simulink model "fw_io_in_hw"  (R2026b)
settings: Solver=VariableStepAuto
undefined symbols (not defined in the file or in its folder): CAN, diff, FD, P, Ts
libraries: simulink x40, stmutilitieslib x5, stm32blockslib x3, stm32h7xxblockslib x2, stm32f4xxblockslib x1, stm32IMUsensorslib x1
settings Model: Creator=aomar  LastModifiedBy=aomar

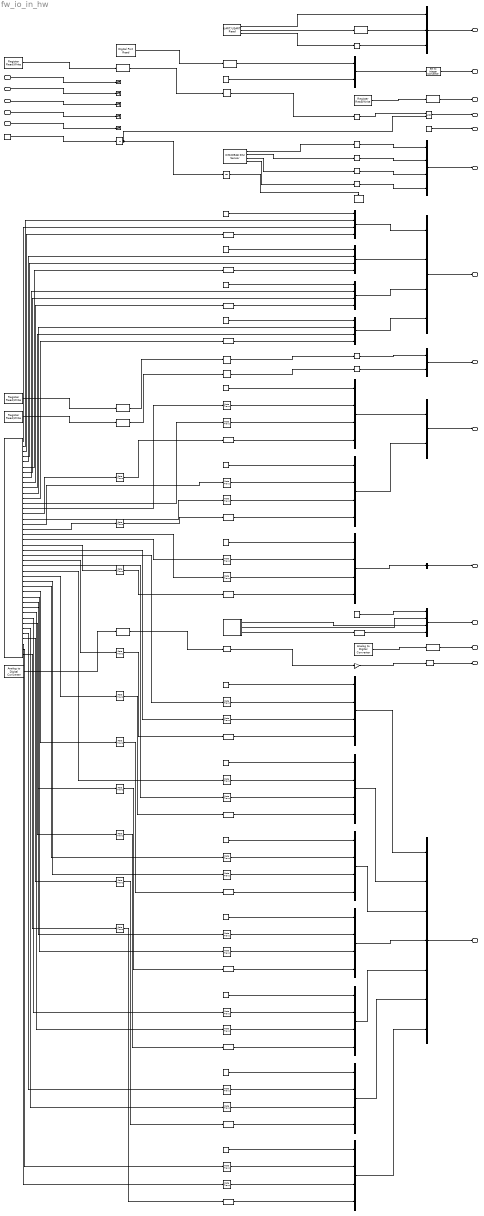
== system fw_io_in_hw ==
  in1k : Inport  OutDataTypeStr=Bus: Bus_McuIn1k  SampleTime=Ts.base
  in5 : Inport  Port=2  OutDataTypeStr=Bus: Bus_McuIn5  SampleTime=Ts.imu
  in10 : Inport  Port=3  OutDataTypeStr=Bus: Bus_McuIn10  SampleTime=Ts.ctrl
  in50 : Inport  Port=4  OutDataTypeStr=Bus: Bus_McuIn50  SampleTime=Ts.comm
  in100 : Inport  Port=5  OutDataTypeStr=Bus: Bus_McuIn100  SampleTime=Ts.hk
  ADC1_Conv : stm32h7xxblockslib/Analog to Digital Converter  ADCModule=ADC1  ConversionGroup=Regular  TriggerMode=Trigger and read  NumberOfConversions=8  EnableBufferConv=off  BufferLength=1  OutputStatus=off  SampleTime=Ts.comm  EnableSimPort=off  hoistedMaskSrc=ECSoC/ECSimCodegen/Analog to Digital Converter
  ADC1_u16 : DataTypeConversion  OutDataTypeStr=uint16  RndMeth=Round
  ADC3_TempSensor : stm32h7xxblockslib/Analog to Digital Converter  ADCModule=ADC3  ConversionGroup=Regular  TriggerMode=Trigger and read  NumberOfConversions=1  EnableBufferConv=off  BufferLength=1  OutputStatus=off  SampleTime=Ts.comm  EnableSimPort=off  hoistedMaskSrc=ECSoC/ECSimCodegen/Analog to Digital Converter
  ADC3_s : DataTypeConversion  OutDataTypeStr=single  RndMeth=Round
  BO1 : simulink/Logic and Bit Operations/Compare To Zero  relop=~=  OutDataTypeStr=boolean
  BO1_bit : simulink/Logic and Bit Operations/Bitwise Operator  logicop=AND  UseBitMask=on  BitMask=2^P.electronics.hw.fdcan_psr_bo_bit  BitMaskRealWorld=Stored Integer
  BO2 : simulink/Logic and Bit Operations/Compare To Zero  relop=~=  OutDataTypeStr=boolean
  BO2_bit : simulink/Logic and Bit Operations/Bitwise Operator  logicop=AND  UseBitMask=on  BitMask=2^P.electronics.hw.fdcan_psr_bo_bit  BitMaskRealWorld=Stored Integer
  BO_vec : Concatenate
  Bms_BC : BusCreator  Inputs=7  OutDataTypeStr=Bus: Bus_Can1_Bms  NonVirtualBus=on
      settings: InheritFromInputs=off
  Boot_false : Constant  Value=false  OutDataTypeStr=boolean  SampleTime=Ts.base
  CAN1_RX : Subsystem  TreatAsAtomicUnit=on  SystemSampleTime=Ts.ctrl
  CAN2_RX : Subsystem  TreatAsAtomicUnit=on  SystemSampleTime=Ts.comm
  DI_GPIOF : stm32f4xxblockslib/Digital Port Read  PortName=GPIOF  PinNumber=[0:13]  ReadOperation=on  IOAsArray=on  SampleTime=Ts.base  EnableSimPort=off  hoistedMaskSrc=ECSoC/ECSimCodegen/Digital Port Read
      settings: LibrarySourceBlock=stm32h7xxblockslib/Digital Port Read
  DI_bits : Concatenate
  DI_bool : DataTypeConversion  OutDataTypeStr=boolean  RndMeth=Round
  DI_pad : Constant  Value=false(1,16-P.electronics.hw.di_pins)  OutDataTypeStr=boolean  SampleTime=Ts.base
  DI_word : simulink/Logic and Bit Operations/Bit to Integer Converter  nbits=16  bitOrder=LSB first  signedOutputValues=Unsigned  outDtype=uint16  outDtypeSigned=Inherit via internal rule
      settings: LibrarySourceBlock=|
      | commutil2/Bit to Integer
      | Converter
  Esc_fast_BC : BusCreator  Inputs=4  OutDataTypeStr=Bus: Bus_Can1_EscFast  NonVirtualBus=on
      settings: InheritFromInputs=off
  Esc_slow_BC : BusCreator  Inputs=2  OutDataTypeStr=Bus: Bus_Can1_EscSlow  NonVirtualBus=on
      settings: InheritFromInputs=off
  FDCAN1_PSR : stmutilitieslib/Register Read//Write  Description=INTENDED (set in the T17 board setup): tgtHW 'STM32H7xx Based', devID 'STM32H743', regGrpName 'FDCAN1', regName 'PSR', opCode 'Read'.  tgtHW=STM32F4xx Based  devID=STM32F401  regGrpName=ADC_Common  regName=CSR  accessMode=Specified bits  opCode=Read  bitsToBeProcessed={ [ 15, 0 ] }  bitFields={'on','All';'off','OVR3';'off','STRT3';'off','JSTRT3';'off','JEOC3';'off','EOC3';'off','AWD3';'off','OVR2';'off','STRT2';'off','JSTRT2';'off','JEOC2';'off','EOC2';'off','AWD2';'off','OVR1';'off','STRT1';'off','JSTRT1';'off','JEOC1';'off','EOC1';'off','AWD1'}  SampleTime=1
  FDCAN2_PSR : stmutilitieslib/Register Read//Write  Description=INTENDED (set in the T17 board setup): tgtHW 'STM32H7xx Based', devID 'STM32H743', regGrpName 'FDCAN2', regName 'PSR', opCode 'Read'.  tgtHW=STM32F4xx Based  devID=STM32F401  regGrpName=ADC_Common  regName=CSR  accessMode=Specified bits  opCode=Read  bitsToBeProcessed={ [ 15, 0 ] }  bitFields={'on','All';'off','OVR3';'off','STRT3';'off','JSTRT3';'off','JEOC3';'off','EOC3';'off','AWD3';'off','OVR2';'off','STRT2';'off','JSTRT2';'off','JEOC2';'off','EOC2';'off','AWD2';'off','OVR1';'off','STRT1';'off','JSTRT1';'off','JEOC1';'off','EOC1';'off','AWD1'}  SampleTime=1
  First_tick : UnitDelay  InitialCondition=true  SampleTime=Ts.base
  Frame_alarm : BusCreator  Inputs=4  OutDataTypeStr=Bus: Bus_CanFrame8  NonVirtualBus=on
      settings: InheritFromInputs=off
  Frame_cells : BusCreator  Inputs=4  OutDataTypeStr=Bus: Bus_CanFrame8  NonVirtualBus=on
      settings: InheritFromInputs=off
  Frame_comp_cmd : BusCreator  Inputs=4  OutDataTypeStr=Bus: Bus_CanFrame64  NonVirtualBus=on
      settings: InheritFromInputs=off
  Frame_fb1_L : BusCreator  Inputs=4  OutDataTypeStr=Bus: Bus_CanFrame8  NonVirtualBus=on
      settings: InheritFromInputs=off
  Frame_fb1_R : BusCreator  Inputs=4  OutDataTypeStr=Bus: Bus_CanFrame8  NonVirtualBus=on
      settings: InheritFromInputs=off
  Frame_fb2_L : BusCreator  Inputs=4  OutDataTypeStr=Bus: Bus_CanFrame8  NonVirtualBus=on
      settings: InheritFromInputs=off
  Frame_fb2_R : BusCreator  Inputs=4  OutDataTypeStr=Bus: Bus_CanFrame8  NonVirtualBus=on
      settings: InheritFromInputs=off
  Frame_fb3_L : BusCreator  Inputs=4  OutDataTypeStr=Bus: Bus_CanFrame8  NonVirtualBus=on
      settings: InheritFromInputs=off
  Frame_fb3_R : BusCreator  Inputs=4  OutDataTypeStr=Bus: Bus_CanFrame8  NonVirtualBus=on
      settings: InheritFromInputs=off
  Frame_impl_fb : BusCreator  Inputs=4  OutDataTypeStr=Bus: Bus_CanFrame8  NonVirtualBus=on
      settings: InheritFromInputs=off
  Frame_limits : BusCreator  Inputs=4  OutDataTypeStr=Bus: Bus_CanFrame8  NonVirtualBus=on
      settings: InheritFromInputs=off
  Frame_power : BusCreator  Inputs=4  OutDataTypeStr=Bus: Bus_CanFrame8  NonVirtualBus=on
      settings: InheritFromInputs=off
  Frame_soc : BusCreator  Inputs=4  OutDataTypeStr=Bus: Bus_CanFrame8  NonVirtualBus=on
      settings: InheritFromInputs=off
  Frame_state : BusCreator  Inputs=4  OutDataTypeStr=Bus: Bus_CanFrame8  NonVirtualBus=on
      settings: InheritFromInputs=off
  Frame_vit : BusCreator  Inputs=4  OutDataTypeStr=Bus: Bus_CanFrame8  NonVirtualBus=on
      settings: InheritFromInputs=off
  ICM20948 : stm32IMUsensorslib/ICM20948 IMU Sensor  I2CModule=I2C1  I2CAddress=0x69  BitRate=400000  EnableDRDY=off  InterruptType=Active high  IsActiveAccel=on  IsActiveGyro=on  IsActiveMag=on  IsActiveTemp=on  IsActiveStatus=off  IsActiveTimeStamp=off  AccelerometerRange=+/-4g  AccelerometerODR=1125  AccelerometerBW=23.9 Hz  GyroscopeRange=+/-500 dps  GyroscopeODR=1125  GyroscopeBW=23.9 Hz  MagnetometerODR=100 Hz  TemperatureBW=34.1 Hz  DataType=single  SampleTime=Ts.imu  QueueSizeFactor=3
  IWDG1RSTF : simulink/Logic and Bit Operations/Bitwise Operator  logicop=AND  UseBitMask=on  BitMask=2^P.electronics.hw.rcc_rsr_iwdg1rstf_bit  BitMaskRealWorld=Stored Integer
  Id_alarm : Constant  Value=P.electronics.can.id.bms_alarm  OutDataTypeStr=uint32  SampleTime=Ts.hk
  Id_cells : Constant  Value=P.electronics.can.id.bms_cells  OutDataTypeStr=uint32  SampleTime=Ts.hk
  Id_comp_cmd : Constant  Value=P.electronics.can.id.comp_cmd  OutDataTypeStr=uint32  SampleTime=Ts.comm
  Id_fb1_L : Constant  Value=P.drive.can.id_fb1+1  OutDataTypeStr=uint32  SampleTime=Ts.ctrl
  Id_fb1_R : Constant  Value=P.drive.can.id_fb1+2  OutDataTypeStr=uint32  SampleTime=Ts.ctrl
  Id_fb2_L : Constant  Value=P.drive.can.id_fb2+1  OutDataTypeStr=uint32  SampleTime=Ts.comm
  Id_fb2_R : Constant  Value=P.drive.can.id_fb2+2  OutDataTypeStr=uint32  SampleTime=Ts.comm
  Id_fb3_L : Constant  Value=P.drive.can.id_fb3+1  OutDataTypeStr=uint32  SampleTime=Ts.ctrl
  Id_fb3_R : Constant  Value=P.drive.can.id_fb3+2  OutDataTypeStr=uint32  SampleTime=Ts.ctrl
  Id_impl_fb : Constant  Value=P.electronics.can.id.impl_fb  OutDataTypeStr=uint32  SampleTime=Ts.comm
  Id_limits : Constant  Value=P.electronics.can.id.bms_limits  OutDataTypeStr=uint32  SampleTime=Ts.hk
  Id_power : Constant  Value=P.electronics.can.id.bms_power  OutDataTypeStr=uint32  SampleTime=Ts.hk
  Id_soc : Constant  Value=P.electronics.can.id.bms_soc  OutDataTypeStr=uint32  SampleTime=Ts.hk
  Id_state : Constant  Value=P.electronics.can.id.bms_state  OutDataTypeStr=uint32  SampleTime=Ts.hk
  Id_vit : Constant  Value=P.electronics.can.id.bms_vit  OutDataTypeStr=uint32  SampleTime=Ts.hk
  Impl_BC : BusCreator  Inputs=1  OutDataTypeStr=Bus: Bus_Can1_Impl  NonVirtualBus=on
      settings: InheritFromInputs=off
  Imu_BC : BusCreator  Inputs=4  OutDataTypeStr=Bus: Bus_ImuRaw  NonVirtualBus=on
      settings: InheritFromInputs=off
  Imu_vec{1..4} (4 alike) : Reshape
  New_alarm : simulink/Logic and Bit Operations/Detect Change  vinit=0  OutDataTypeStr=boolean
  New_cells : simulink/Logic and Bit Operations/Detect Change  vinit=0  OutDataTypeStr=boolean
  New_comp_cmd : simulink/Logic and Bit Operations/Detect Change  vinit=0  OutDataTypeStr=boolean
  New_fb1_L : simulink/Logic and Bit Operations/Detect Change  vinit=0  OutDataTypeStr=boolean
  New_fb1_R : simulink/Logic and Bit Operations/Detect Change  vinit=0  OutDataTypeStr=boolean
  New_fb2_L : simulink/Logic and Bit Operations/Detect Change  vinit=0  OutDataTypeStr=boolean
  New_fb2_R : simulink/Logic and Bit Operations/Detect Change  vinit=0  OutDataTypeStr=boolean
  New_fb3_L : simulink/Logic and Bit Operations/Detect Change  vinit=0  OutDataTypeStr=boolean
  New_fb3_R : simulink/Logic and Bit Operations/Detect Change  vinit=0  OutDataTypeStr=boolean
  New_impl_fb : simulink/Logic and Bit Operations/Detect Change  vinit=0  OutDataTypeStr=boolean
  New_limits : simulink/Logic and Bit Operations/Detect Change  vinit=0  OutDataTypeStr=boolean
  New_power : simulink/Logic and Bit Operations/Detect Change  vinit=0  OutDataTypeStr=boolean
  New_soc : simulink/Logic and Bit Operations/Detect Change  vinit=0  OutDataTypeStr=boolean
  New_state : simulink/Logic and Bit Operations/Detect Change  vinit=0  OutDataTypeStr=boolean
  New_vit : simulink/Logic and Bit Operations/Detect Change  vinit=0  OutDataTypeStr=boolean
  No_inject : Constant  Value=0  OutDataTypeStr=uint32  SampleTime=Ts.base
  PSR1_u32 : DataTypeConversion  OutDataTypeStr=uint32  RndMeth=Round
  PSR2_u32 : DataTypeConversion  OutDataTypeStr=uint32  RndMeth=Round
  RCC_RSR : stmutilitieslib/Register Read//Write  Description=INTENDED (set in the T17 board setup): tgtHW 'STM32H7xx Based', devID 'STM32H743', regGrpName 'RCC', regName 'RSR', opCode 'Read'.  tgtHW=STM32F4xx Based  devID=STM32F401  regGrpName=ADC_Common  regName=CSR  accessMode=Specified bits  opCode=Read  bitsToBeProcessed={ [ 15, 0 ] }  bitFields={'on','All';'off','OVR3';'off','STRT3';'off','JSTRT3';'off','JEOC3';'off','EOC3';'off','AWD3';'off','OVR2';'off','STRT2';'off','JSTRT2';'off','JEOC2';'off','EOC2';'off','AWD2';'off','OVR1';'off','STRT1';'off','JSTRT1';'off','JEOC1';'off','EOC1';'off','AWD1'}  SampleTime=1
  RMVF_write : Subsystem
  RSR_u32 : DataTypeConversion  OutDataTypeStr=uint32  RndMeth=Round
  RT_alarm_1 : RateTransition  OutPortSampleTime=Ts.hk
  RT_alarm_2 : RateTransition  OutPortSampleTime=Ts.hk
  RT_alarm_3 : RateTransition  OutPortSampleTime=Ts.hk
  RT_cells_1 : RateTransition  OutPortSampleTime=Ts.hk
  RT_cells_2 : RateTransition  OutPortSampleTime=Ts.hk
  RT_cells_3 : RateTransition  OutPortSampleTime=Ts.hk
  RT_fb2_L_1 : RateTransition  OutPortSampleTime=Ts.comm
  RT_fb2_L_2 : RateTransition  OutPortSampleTime=Ts.comm
  RT_fb2_L_3 : RateTransition  OutPortSampleTime=Ts.comm
  RT_fb2_R_1 : RateTransition  OutPortSampleTime=Ts.comm
  RT_fb2_R_2 : RateTransition  OutPortSampleTime=Ts.comm
  RT_fb2_R_3 : RateTransition  OutPortSampleTime=Ts.comm
  RT_impl_fb_1 : RateTransition  OutPortSampleTime=Ts.comm
  RT_impl_fb_2 : RateTransition  OutPortSampleTime=Ts.comm
  RT_impl_fb_3 : RateTransition  OutPortSampleTime=Ts.comm
  RT_limits_1 : RateTransition  OutPortSampleTime=Ts.hk
  RT_limits_2 : RateTransition  OutPortSampleTime=Ts.hk
  RT_limits_3 : RateTransition  OutPortSampleTime=Ts.hk
  RT_power_1 : RateTransition  OutPortSampleTime=Ts.hk
  RT_power_2 : RateTransition  OutPortSampleTime=Ts.hk
  RT_power_3 : RateTransition  OutPortSampleTime=Ts.hk
  RT_soc_1 : RateTransition  OutPortSampleTime=Ts.hk
  RT_soc_2 : RateTransition  OutPortSampleTime=Ts.hk
  RT_soc_3 : RateTransition  OutPortSampleTime=Ts.hk
  RT_state_1 : RateTransition  OutPortSampleTime=Ts.hk
  RT_state_2 : RateTransition  OutPortSampleTime=Ts.hk
  RT_state_3 : RateTransition  OutPortSampleTime=Ts.hk
  RT_vit_1 : RateTransition  OutPortSampleTime=Ts.hk
  RT_vit_2 : RateTransition  OutPortSampleTime=Ts.hk
  RT_vit_3 : RateTransition  OutPortSampleTime=Ts.hk
  Reset_at_boot : Logic  AllPortsSameDT=off  OutDataTypeStr=boolean
  Rst_seen : simulink/Logic and Bit Operations/Compare To Zero  relop=~=  OutDataTypeStr=boolean
  SBUS_UART : stm32blockslib/UART//USART Read  UARTModule=USART2  DataType=uint8  DataLength=32  BlockingMode=off  BlockingTimeout=0.1  OutputLength=on  OutputStatus=on  SampleTime=Ts.base
      settings: LibrarySourceBlock=stm32h7xxblockslib/UART//USART Read
  Sbus_BC : BusCreator  Inputs=3  OutDataTypeStr=Bus: Bus_SbusStream  NonVirtualBus=on
      settings: InheritFromInputs=off
  Second_tick : UnitDelay  InitialCondition=false  SampleTime=Ts.base
  TIM2_CNT : stmutilitieslib/Register Read//Write  Description=INTENDED (set in the T17 board setup): tgtHW 'STM32H7xx Based', devID 'STM32H743', regGrpName 'TIM2', regName 'CNT', opCode 'Read'.  tgtHW=STM32F4xx Based  devID=STM32F401  regGrpName=ADC_Common  regName=CSR  accessMode=Specified bits  opCode=Read  bitsToBeProcessed={ [ 15, 0 ] }  bitFields={'on','All';'off','OVR3';'off','STRT3';'off','JSTRT3';'off','JEOC3';'off','EOC3';'off','AWD3';'off','OVR2';'off','STRT2';'off','JSTRT2';'off','JEOC2';'off','EOC2';'off','AWD2';'off','OVR1';'off','STRT1';'off','JSTRT1';'off','JEOC1';'off','EOC1';'off','AWD1'}  SampleTime=1
  TS_T1 : Bias  Bias=P.electronics.adc.ts_cal_T(1)  SaturateOnIntegerOverflow=off
  TS_c1 : Bias  Bias=-P.electronics.adc.ts_cal_cnt(1)  SaturateOnIntegerOverflow=off
  TS_slope : Gain  Gain=diff(P.electronics.adc.ts_cal_T)/diff(P.electronics.adc.ts_cal_cnt)
  T_in{5,10,50,100} (4 alike) : Terminator
  T_in1k : Terminator
  T_us_u32 : DataTypeConversion  OutDataTypeStr=uint32  RndMeth=Round
  Uart_err : simulink/Logic and Bit Operations/Compare To Zero  relop=~=  OutDataTypeStr=boolean
  Uart_len : DataTypeConversion  OutDataTypeStr=uint8  RndMeth=Round
  sbus : Outport  OutDataTypeStr=Bus: Bus_SbusStream
  di_word : Outport  Port=2  OutDataTypeStr=uint16
  t_us : Outport  Port=3  OutDataTypeStr=uint32
  reset_flag : Outport  Port=4  OutDataTypeStr=boolean
  fault_inject : Outport  Port=5  OutDataTypeStr=uint32
  imu : Outport  Port=6  OutDataTypeStr=Bus: Bus_ImuRaw
  can1_esc : Outport  Port=7  OutDataTypeStr=Bus: Bus_Can1_EscFast
  busoff : Outport  Port=8  OutDataTypeStr=boolean
  can1_escslow : Outport  Port=9  OutDataTypeStr=Bus: Bus_Can1_EscSlow
  can1_impl : Outport  Port=10  OutDataTypeStr=Bus: Bus_Can1_Impl
  can2_comp : Outport  Port=11  OutDataTypeStr=Bus: Bus_CanFrame64
  adc_raw : Outport  Port=12  OutDataTypeStr=uint16
  mcu_temp_degC : Outport  Port=13  OutDataTypeStr=single
  can1_bms : Outport  Port=14  OutDataTypeStr=Bus: Bus_Can1_Bms
  wires:
  in1k/1 -> T_in1k/1  "in1k"
  in5/1 -> T_in5/1  "in5"
  in10/1 -> T_in10/1  "in10"
  in50/1 -> T_in50/1  "in50"
  in100/1 -> T_in100/1  "in100"
  Boot_false/1 -> First_tick/1  "Boot_false"
  RCC_RSR/1 -> RSR_u32/1  "RCC_RSR"
  FDCAN1_PSR/1 -> PSR1_u32/1  "FDCAN1_PSR"
  FDCAN2_PSR/1 -> PSR2_u32/1  "FDCAN2_PSR"
  CAN1_RX/1(data_fb1_L) -> Frame_fb1_L/3  "data"
  CAN1_RX/2(len_fb1_L) -> Frame_fb1_L/2  "len"
  CAN1_RX/3(cnt_fb1_L) -> New_fb1_L/1  "cnt_fb1_L"
  CAN1_RX/4(data_fb1_R) -> Frame_fb1_R/3  "data"
  CAN1_RX/5(len_fb1_R) -> Frame_fb1_R/2  "len"
  CAN1_RX/6(cnt_fb1_R) -> New_fb1_R/1  "cnt_fb1_R"
  CAN1_RX/7(data_fb3_L) -> Frame_fb3_L/3  "data"
  CAN1_RX/8(len_fb3_L) -> Frame_fb3_L/2  "len"
  CAN1_RX/9(cnt_fb3_L) -> New_fb3_L/1  "cnt_fb3_L"
  CAN1_RX/10(data_fb3_R) -> Frame_fb3_R/3  "data"
  CAN1_RX/11(len_fb3_R) -> Frame_fb3_R/2  "len"
  CAN1_RX/12(cnt_fb3_R) -> New_fb3_R/1  "cnt_fb3_R"
  CAN1_RX/13(data_fb2_L) -> RT_fb2_L_1/1  "CAN1_RX_13"
  CAN1_RX/14(len_fb2_L) -> RT_fb2_L_2/1  "CAN1_RX_14"
  CAN1_RX/15(cnt_fb2_L) -> RT_fb2_L_3/1  "CAN1_RX_15"
  CAN1_RX/16(data_fb2_R) -> RT_fb2_R_1/1  "CAN1_RX_16"
  CAN1_RX/17(len_fb2_R) -> RT_fb2_R_2/1  "CAN1_RX_17"
  CAN1_RX/18(cnt_fb2_R) -> RT_fb2_R_3/1  "CAN1_RX_18"
  CAN1_RX/19(data_impl_fb) -> RT_impl_fb_1/1  "CAN1_RX_19"
  CAN1_RX/20(len_impl_fb) -> RT_impl_fb_2/1  "CAN1_RX_20"
  CAN1_RX/21(cnt_impl_fb) -> RT_impl_fb_3/1  "CAN1_RX_21"
  CAN1_RX/22(data_limits) -> RT_limits_1/1  "CAN1_RX_22"
  CAN1_RX/23(len_limits) -> RT_limits_2/1  "CAN1_RX_23"
  CAN1_RX/24(cnt_limits) -> RT_limits_3/1  "CAN1_RX_24"
  CAN1_RX/25(data_soc) -> RT_soc_1/1  "CAN1_RX_25"
  CAN1_RX/26(len_soc) -> RT_soc_2/1  "CAN1_RX_26"
  CAN1_RX/27(cnt_soc) -> RT_soc_3/1  "CAN1_RX_27"
  CAN1_RX/28(data_vit) -> RT_vit_1/1  "CAN1_RX_28"
  CAN1_RX/29(len_vit) -> RT_vit_2/1  "CAN1_RX_29"
  CAN1_RX/30(cnt_vit) -> RT_vit_3/1  "CAN1_RX_30"
  CAN1_RX/31(data_alarm) -> RT_alarm_1/1  "CAN1_RX_31"
  CAN1_RX/32(len_alarm) -> RT_alarm_2/1  "CAN1_RX_32"
  CAN1_RX/33(cnt_alarm) -> RT_alarm_3/1  "CAN1_RX_33"
  CAN1_RX/34(data_cells) -> RT_cells_1/1  "CAN1_RX_34"
  CAN1_RX/35(len_cells) -> RT_cells_2/1  "CAN1_RX_35"
  CAN1_RX/36(cnt_cells) -> RT_cells_3/1  "CAN1_RX_36"
  CAN1_RX/37(data_state) -> RT_state_1/1  "CAN1_RX_37"
  CAN1_RX/38(len_state) -> RT_state_2/1  "CAN1_RX_38"
  CAN1_RX/39(cnt_state) -> RT_state_3/1  "CAN1_RX_39"
  CAN1_RX/40(data_power) -> RT_power_1/1  "CAN1_RX_40"
  CAN1_RX/41(len_power) -> RT_power_2/1  "CAN1_RX_41"
  CAN1_RX/42(cnt_power) -> RT_power_3/1  "CAN1_RX_42"
  ADC3_TempSensor/1 -> ADC3_s/1  "ADC3_TempSensor"
  First_tick/1 -> Second_tick/1, Reset_at_boot/2  "first_tick"
  RT_fb2_L_3/1 -> New_fb2_L/1  "cnt_fb2_L"
  RT_fb2_R_3/1 -> New_fb2_R/1  "cnt_fb2_R"
  RT_impl_fb_3/1 -> New_impl_fb/1  "cnt_impl_fb"
  RT_limits_3/1 -> New_limits/1  "cnt_limits"
  RT_soc_3/1 -> New_soc/1  "cnt_soc"
  RT_vit_3/1 -> New_vit/1  "cnt_vit"
  RT_alarm_3/1 -> New_alarm/1  "cnt_alarm"
  RT_cells_3/1 -> New_cells/1  "cnt_cells"
  RT_state_3/1 -> New_state/1  "cnt_state"
  RT_power_3/1 -> New_power/1  "cnt_power"
  RSR_u32/1 -> IWDG1RSTF/1  "RSR_u32"
  PSR1_u32/1 -> BO1_bit/1  "PSR1_u32"
  PSR2_u32/1 -> BO2_bit/1  "PSR2_u32"
  ADC3_s/1 -> TS_c1/1  "ADC3_s"
  DI_GPIOF/1 -> DI_bool/1  "DI_GPIOF"
  DI_pad/1 -> DI_bits/2  "DI_pad"
  Id_fb1_L/1 -> Frame_fb1_L/1  "id"
  Id_fb1_R/1 -> Frame_fb1_R/1  "id"
  Id_fb3_L/1 -> Frame_fb3_L/1  "id"
  Id_fb3_R/1 -> Frame_fb3_R/1  "id"
  Id_fb2_L/1 -> Frame_fb2_L/1  "id"
  Id_fb2_R/1 -> Frame_fb2_R/1  "id"
  Id_impl_fb/1 -> Frame_impl_fb/1  "id"
  Id_limits/1 -> Frame_limits/1  "id"
  Id_soc/1 -> Frame_soc/1  "id"
  Id_vit/1 -> Frame_vit/1  "id"
  Id_alarm/1 -> Frame_alarm/1  "id"
  Id_cells/1 -> Frame_cells/1  "id"
  Id_state/1 -> Frame_state/1  "id"
  Id_power/1 -> Frame_power/1  "id"
  Second_tick/1 -> RMVF_write/Enable  "second_tick"
  IWDG1RSTF/1 -> Rst_seen/1  "IWDG1RSTF"
  BO1_bit/1 -> BO1/1  "BO1_bit"
  BO2_bit/1 -> BO2/1  "BO2_bit"
  RT_fb2_L_2/1 -> Frame_fb2_L/2  "len"
  RT_fb2_L_1/1 -> Frame_fb2_L/3  "data"
  RT_fb2_R_2/1 -> Frame_fb2_R/2  "len"
  RT_fb2_R_1/1 -> Frame_fb2_R/3  "data"
  RT_impl_fb_2/1 -> Frame_impl_fb/2  "len"
  RT_impl_fb_1/1 -> Frame_impl_fb/3  "data"
  TS_c1/1 -> TS_slope/1  "TS_c1"
  RT_limits_2/1 -> Frame_limits/2  "len"
  RT_limits_1/1 -> Frame_limits/3  "data"
  RT_soc_2/1 -> Frame_soc/2  "len"
  RT_soc_1/1 -> Frame_soc/3  "data"
  RT_vit_2/1 -> Frame_vit/2  "len"
  RT_vit_1/1 -> Frame_vit/3  "data"
  RT_alarm_2/1 -> Frame_alarm/2  "len"
  RT_alarm_1/1 -> Frame_alarm/3  "data"
  RT_cells_2/1 -> Frame_cells/2  "len"
  RT_cells_1/1 -> Frame_cells/3  "data"
  RT_state_2/1 -> Frame_state/2  "len"
  RT_state_1/1 -> Frame_state/3  "data"
  RT_power_2/1 -> Frame_power/2  "len"
  RT_power_1/1 -> Frame_power/3  "data"
  New_fb1_L/1 -> Frame_fb1_L/4  "valid"
  New_fb1_R/1 -> Frame_fb1_R/4  "valid"
  New_fb3_L/1 -> Frame_fb3_L/4  "valid"
  New_fb3_R/1 -> Frame_fb3_R/4  "valid"
  New_fb2_L/1 -> Frame_fb2_L/4  "valid"
  New_fb2_R/1 -> Frame_fb2_R/4  "valid"
  New_impl_fb/1 -> Frame_impl_fb/4  "valid"
  New_limits/1 -> Frame_limits/4  "valid"
  New_soc/1 -> Frame_soc/4  "valid"
  New_vit/1 -> Frame_vit/4  "valid"
  New_alarm/1 -> Frame_alarm/4  "valid"
  New_cells/1 -> Frame_cells/4  "valid"
  New_state/1 -> Frame_state/4  "valid"
  New_power/1 -> Frame_power/4  "valid"
  DI_bool/1 -> DI_bits/1  "DI_bool"
  SBUS_UART/1 -> Sbus_BC/1  "bytes"
  SBUS_UART/2 -> Uart_len/1  "SBUS_UART_2"
  SBUS_UART/3 -> Uart_err/1  "SBUS_UART_3"
  CAN2_RX/1(data_comp_cmd) -> Frame_comp_cmd/3  "data"
  CAN2_RX/2(len_comp_cmd) -> Frame_comp_cmd/2  "len"
  CAN2_RX/3(cnt_comp_cmd) -> New_comp_cmd/1  "cnt_comp_cmd"
  ICM20948/1 -> Imu_vec1/1  "ICM20948_1"
  ICM20948/2 -> Imu_vec2/1  "ICM20948_2"
  ICM20948/3 -> Imu_vec3/1  "ICM20948_3"
  ICM20948/4 -> Imu_vec4/1  "ICM20948_4"
  DI_bits/1 -> DI_word/1  "DI_bits"
  Frame_fb1_L/1 -> Esc_fast_BC/1  "fb1_L"
  Frame_fb1_R/1 -> Esc_fast_BC/2  "fb1_R"
  Frame_fb3_L/1 -> Esc_fast_BC/3  "fb3_L"
  Frame_fb3_R/1 -> Esc_fast_BC/4  "fb3_R"
  Frame_fb2_L/1 -> Esc_slow_BC/1  "fb2_L"
  Frame_fb2_R/1 -> Esc_slow_BC/2  "fb2_R"
  Frame_impl_fb/1 -> Impl_BC/1  "impl_fb"
  Frame_limits/1 -> Bms_BC/1  "limits"
  Frame_soc/1 -> Bms_BC/2  "soc"
  Frame_vit/1 -> Bms_BC/3  "vit"
  Frame_alarm/1 -> Bms_BC/4  "alarm"
  Frame_cells/1 -> Bms_BC/5  "cells"
  Frame_state/1 -> Bms_BC/6  "state"
  Frame_power/1 -> Bms_BC/7  "power"
  Uart_err/1 -> Sbus_BC/3  "uart_err"
  Rst_seen/1 -> Reset_at_boot/1  "Rst_seen"
  Imu_vec1/1 -> Imu_BC/1  "Acceleration"
  Imu_vec2/1 -> Imu_BC/2  "AngularRate"
  Imu_vec3/1 -> Imu_BC/3  "MagneticField"
  Imu_vec4/1 -> Imu_BC/4  "Temperature"
  BO1/1 -> BO_vec/1  "can1_busoff"
  BO2/1 -> BO_vec/2  "can2_busoff"
  Id_comp_cmd/1 -> Frame_comp_cmd/1  "id"
  TS_slope/1 -> TS_T1/1  "TS_slope"
  New_comp_cmd/1 -> Frame_comp_cmd/4  "valid"
  Uart_len/1 -> Sbus_BC/2  "len"
  TIM2_CNT/1 -> T_us_u32/1  "TIM2_CNT"
  ADC1_Conv/1 -> ADC1_u16/1  "ADC1_Conv"
  Sbus_BC/1 -> sbus/1  "sbus"
  Imu_BC/1 -> imu/1  "imu"
  Esc_fast_BC/1 -> can1_esc/1  "can1_esc"
  BO_vec/1 -> busoff/1  "busoff"
  Esc_slow_BC/1 -> can1_escslow/1  "can1_escslow"
  Impl_BC/1 -> can1_impl/1  "can1_impl"
  Frame_comp_cmd/1 -> can2_comp/1  "can2_comp"
  Bms_BC/1 -> can1_bms/1  "can1_bms"
  Reset_at_boot/1 -> reset_flag/1  "reset_flag"
  No_inject/1 -> fault_inject/1  "fault_inject"
  TS_T1/1 -> mcu_temp_degC/1  "mcu_temp_degC"
  T_us_u32/1 -> t_us/1  "t_us"
  ADC1_u16/1 -> adc_raw/1  "adc_raw"
  DI_word/1 -> di_word/1  "di_word"

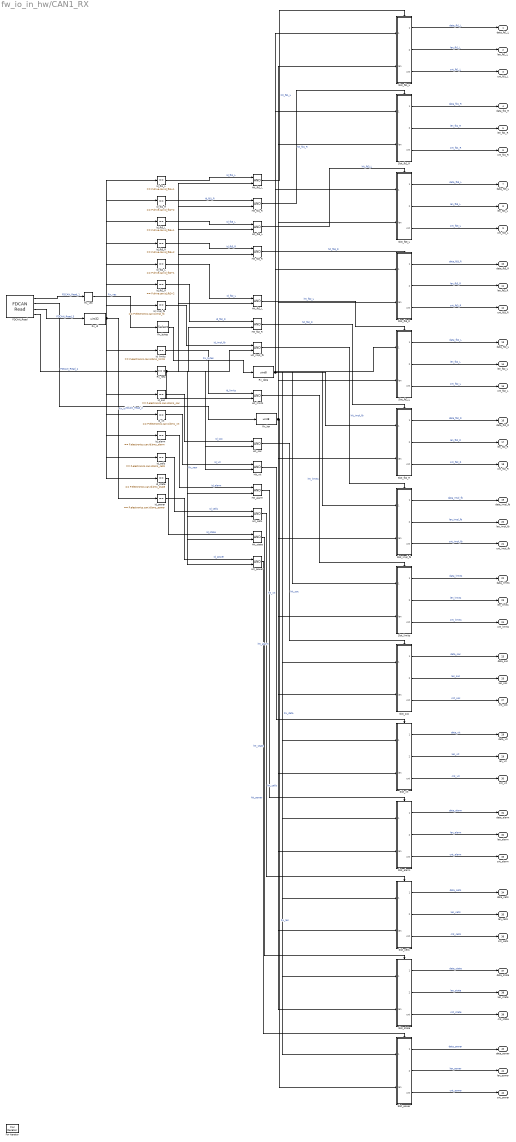
== system fw_io_in_hw/CAN1_RX ==
  FDCAN_Read : stm32blockslib/FDCAN Read  FDCANModule=FDCAN1  BlockMode=Receive  OperationReadMode=Data  OperationWriteMode=Data  ReadSource=FIFO 0  BufferNumber=0  OutputTypeReadMode=Unpacked  DataFormatWriteMode=Raw data  CANFrameType=CAN  IdentifierTypeVia=Dialog  IdentifierType=Standard (11-bit identifier)  IdentifierVia=Inport  Identifier=100  DataLengthVia=Inport  DataLength=64  OutputIdType=off  IsBitRateSwitchingEnabled=off  TransmitRemoteFrame=off  OutputFrameType=off  OutputBRS=off  OutputRemoteFrame=off  OutputTxFifoLevel=off  OutputRxFifoLevel=off  OutputStatus=on  Timeout=0.001  SampleTime=-1
      settings: LibrarySourceBlock=stm32h7xxblockslib/FDCAN Read
  For Iterator : ForIterator  IterationLimit=P.electronics.hw.can1_rx_iter  ShowIterationPort=off
  Hit_alarm : Logic  AllPortsSameDT=off  OutDataTypeStr=boolean
  Hit_cells : Logic  AllPortsSameDT=off  OutDataTypeStr=boolean
  Hit_fb1_L : Logic  AllPortsSameDT=off  OutDataTypeStr=boolean
  Hit_fb1_R : Logic  AllPortsSameDT=off  OutDataTypeStr=boolean
  Hit_fb2_L : Logic  AllPortsSameDT=off  OutDataTypeStr=boolean
  Hit_fb2_R : Logic  AllPortsSameDT=off  OutDataTypeStr=boolean
  Hit_fb3_L : Logic  AllPortsSameDT=off  OutDataTypeStr=boolean
  Hit_fb3_R : Logic  AllPortsSameDT=off  OutDataTypeStr=boolean
  Hit_impl_fb : Logic  AllPortsSameDT=off  OutDataTypeStr=boolean
  Hit_limits : Logic  AllPortsSameDT=off  OutDataTypeStr=boolean
  Hit_power : Logic  AllPortsSameDT=off  OutDataTypeStr=boolean
  Hit_soc : Logic  AllPortsSameDT=off  OutDataTypeStr=boolean
  Hit_state : Logic  AllPortsSameDT=off  OutDataTypeStr=boolean
  Hit_vit : Logic  AllPortsSameDT=off  OutDataTypeStr=boolean
  Id_alarm : simulink/Logic and Bit Operations/Compare To Constant  relop===  const=P.electronics.can.id.bms_alarm  OutDataTypeStr=boolean
  Id_cells : simulink/Logic and Bit Operations/Compare To Constant  relop===  const=P.electronics.can.id.bms_cells  OutDataTypeStr=boolean
  Id_fb1_L : simulink/Logic and Bit Operations/Compare To Constant  relop===  const=P.drive.can.id_fb1+1  OutDataTypeStr=boolean
  Id_fb1_R : simulink/Logic and Bit Operations/Compare To Constant  relop===  const=P.drive.can.id_fb1+2  OutDataTypeStr=boolean
  Id_fb2_L : simulink/Logic and Bit Operations/Compare To Constant  relop===  const=P.drive.can.id_fb2+1  OutDataTypeStr=boolean
  Id_fb2_R : simulink/Logic and Bit Operations/Compare To Constant  relop===  const=P.drive.can.id_fb2+2  OutDataTypeStr=boolean
  Id_fb3_L : simulink/Logic and Bit Operations/Compare To Constant  relop===  const=P.drive.can.id_fb3+1  OutDataTypeStr=boolean
  Id_fb3_R : simulink/Logic and Bit Operations/Compare To Constant  relop===  const=P.drive.can.id_fb3+2  OutDataTypeStr=boolean
  Id_impl_fb : simulink/Logic and Bit Operations/Compare To Constant  relop===  const=P.electronics.can.id.impl_fb  OutDataTypeStr=boolean
  Id_limits : simulink/Logic and Bit Operations/Compare To Constant  relop===  const=P.electronics.can.id.bms_limits  OutDataTypeStr=boolean
  Id_power : simulink/Logic and Bit Operations/Compare To Constant  relop===  const=P.electronics.can.id.bms_power  OutDataTypeStr=boolean
  Id_soc : simulink/Logic and Bit Operations/Compare To Constant  relop===  const=P.electronics.can.id.bms_soc  OutDataTypeStr=boolean
  Id_state : simulink/Logic and Bit Operations/Compare To Constant  relop===  const=P.electronics.can.id.bms_state  OutDataTypeStr=boolean
  Id_vit : simulink/Logic and Bit Operations/Compare To Constant  relop===  const=P.electronics.can.id.bms_vit  OutDataTypeStr=boolean
  Rx_bytes : Selector  IndexOptions=Index vector (dialog)  Indices=1:8  OutputSizes=1
  Rx_data : DataTypeConversion  OutDataTypeStr=uint8  RndMeth=Round
  Rx_id : DataTypeConversion  OutDataTypeStr=uint32  RndMeth=Round
  Rx_len : DataTypeConversion  OutDataTypeStr=uint8  RndMeth=Round
  Rx_new : simulink/Logic and Bit Operations/Compare To Zero  relop===  OutDataTypeStr=boolean
  Rx_vec : Reshape
  Slot_alarm : Subsystem
  Slot_cells : Subsystem
  Slot_fb1_L : Subsystem
  Slot_fb1_R : Subsystem
  Slot_fb2_L : Subsystem
  Slot_fb2_R : Subsystem
  Slot_fb3_L : Subsystem
  Slot_fb3_R : Subsystem
  Slot_impl_fb : Subsystem
  Slot_limits : Subsystem
  Slot_power : Subsystem
  Slot_soc : Subsystem
  Slot_state : Subsystem
  Slot_vit : Subsystem
  data_fb1_L : Outport
  len_fb1_L : Outport  Port=2
  cnt_fb1_L : Outport  Port=3
  data_fb1_R : Outport  Port=4
  len_fb1_R : Outport  Port=5
  cnt_fb1_R : Outport  Port=6
  data_fb3_L : Outport  Port=7
  len_fb3_L : Outport  Port=8
  cnt_fb3_L : Outport  Port=9
  data_fb3_R : Outport  Port=10
  len_fb3_R : Outport  Port=11
  cnt_fb3_R : Outport  Port=12
  data_fb2_L : Outport  Port=13
  len_fb2_L : Outport  Port=14
  cnt_fb2_L : Outport  Port=15
  data_fb2_R : Outport  Port=16
  len_fb2_R : Outport  Port=17
  cnt_fb2_R : Outport  Port=18
  data_impl_fb : Outport  Port=19
  len_impl_fb : Outport  Port=20
  cnt_impl_fb : Outport  Port=21
  data_limits : Outport  Port=22
  len_limits : Outport  Port=23
  cnt_limits : Outport  Port=24
  data_soc : Outport  Port=25
  len_soc : Outport  Port=26
  cnt_soc : Outport  Port=27
  data_vit : Outport  Port=28
  len_vit : Outport  Port=29
  cnt_vit : Outport  Port=30
  data_alarm : Outport  Port=31
  len_alarm : Outport  Port=32
  cnt_alarm : Outport  Port=33
  data_cells : Outport  Port=34
  len_cells : Outport  Port=35
  cnt_cells : Outport  Port=36
  data_state : Outport  Port=37
  len_state : Outport  Port=38
  cnt_state : Outport  Port=39
  data_power : Outport  Port=40
  len_power : Outport  Port=41
  cnt_power : Outport  Port=42
  wires:
  FDCAN_Read/1 -> Rx_vec/1  "FDCAN_Read_1"
  FDCAN_Read/2 -> Rx_len/1  "FDCAN_Read_2"
  FDCAN_Read/3 -> Rx_id/1  "FDCAN_Read_3"
  FDCAN_Read/4 -> Rx_new/1  "FDCAN_Read_4"
  Rx_vec/1 -> Rx_bytes/1  "Rx_vec"
  Rx_id/1 -> Id_power/1, Id_state/1, Id_fb1_L/1, Id_cells/1, Id_fb1_R/1, Id_alarm/1, Id_fb3_L/1, Id_vit/1, Id_fb3_R/1, Id_soc/1, Id_fb2_L/1, Id_fb2_R/1, Id_limits/1, Id_impl_fb/1  "Rx_id"
  Id_fb1_L/1 -> Hit_fb1_L/1  "Id_fb1_L"
  Id_fb1_R/1 -> Hit_fb1_R/1  "Id_fb1_R"
  Id_fb3_L/1 -> Hit_fb3_L/1  "Id_fb3_L"
  Id_fb3_R/1 -> Hit_fb3_R/1  "Id_fb3_R"
  Id_fb2_L/1 -> Hit_fb2_L/1  "Id_fb2_L"
  Id_fb2_R/1 -> Hit_fb2_R/1  "Id_fb2_R"
  Id_impl_fb/1 -> Hit_impl_fb/1  "Id_impl_fb"
  Id_limits/1 -> Hit_limits/1  "Id_limits"
  Rx_new/1 -> Hit_power/2, Hit_fb1_L/2, Hit_state/2, Hit_fb1_R/2, Hit_cells/2, Hit_fb3_L/2, Hit_alarm/2, Hit_fb3_R/2, Hit_vit/2, Hit_soc/2, Hit_fb2_L/2, Hit_fb2_R/2, Hit_limits/2, Hit_impl_fb/2  "Rx_new"
  Id_soc/1 -> Hit_soc/1  "Id_soc"
  Id_vit/1 -> Hit_vit/1  "Id_vit"
  Id_alarm/1 -> Hit_alarm/1  "Id_alarm"
  Id_cells/1 -> Hit_cells/1  "Id_cells"
  Id_state/1 -> Hit_state/1  "Id_state"
  Id_power/1 -> Hit_power/1  "Id_power"
  Rx_bytes/1 -> Rx_data/1  "Rx_bytes"
  Hit_fb1_L/1 -> Slot_fb1_L/Enable  "hit_fb1_L"
  Hit_fb1_R/1 -> Slot_fb1_R/Enable  "hit_fb1_R"
  Hit_fb3_L/1 -> Slot_fb3_L/Enable  "hit_fb3_L"
  Hit_fb3_R/1 -> Slot_fb3_R/Enable  "hit_fb3_R"
  Hit_fb2_L/1 -> Slot_fb2_L/Enable  "hit_fb2_L"
  Hit_fb2_R/1 -> Slot_fb2_R/Enable  "hit_fb2_R"
  Hit_impl_fb/1 -> Slot_impl_fb/Enable  "hit_impl_fb"
  Hit_limits/1 -> Slot_limits/Enable  "hit_limits"
  Hit_soc/1 -> Slot_soc/Enable  "hit_soc"
  Hit_vit/1 -> Slot_vit/Enable  "hit_vit"
  Hit_alarm/1 -> Slot_alarm/Enable  "hit_alarm"
  Hit_cells/1 -> Slot_cells/Enable  "hit_cells"
  Hit_state/1 -> Slot_state/Enable  "hit_state"
  Hit_power/1 -> Slot_power/Enable  "hit_power"
  Rx_data/1 -> Slot_power/1(data), Slot_state/1(data), Slot_cells/1(data), Slot_alarm/1(data), Slot_vit/1(data), Slot_fb1_L/1(data), Slot_soc/1(data), Slot_fb1_R/1(data), Slot_limits/1(data), Slot_fb3_L/1(data), Slot_impl_fb/1(data), Slot_fb3_R/1(data), Slot_fb2_R/1(data), Slot_fb2_L/1(data)  "Rx_data"
  Rx_len/1 -> Slot_power/2(len), Slot_state/2(len), Slot_cells/2(len), Slot_alarm/2(len), Slot_vit/2(len), Slot_fb1_L/2(len), Slot_soc/2(len), Slot_fb1_R/2(len), Slot_limits/2(len), Slot_fb3_L/2(len), Slot_impl_fb/2(len), Slot_fb3_R/2(len), Slot_fb2_R/2(len), Slot_fb2_L/2(len)  "Rx_len"
  Slot_fb1_L/1(data_h) -> data_fb1_L/1  "data_fb1_L"
  Slot_fb1_L/2(len_h) -> len_fb1_L/1  "len_fb1_L"
  Slot_fb1_L/3(cnt) -> cnt_fb1_L/1  "cnt_fb1_L"
  Slot_fb1_R/1(data_h) -> data_fb1_R/1  "data_fb1_R"
  Slot_fb1_R/2(len_h) -> len_fb1_R/1  "len_fb1_R"
  Slot_fb1_R/3(cnt) -> cnt_fb1_R/1  "cnt_fb1_R"
  Slot_fb3_L/1(data_h) -> data_fb3_L/1  "data_fb3_L"
  Slot_fb3_L/2(len_h) -> len_fb3_L/1  "len_fb3_L"
  Slot_fb3_L/3(cnt) -> cnt_fb3_L/1  "cnt_fb3_L"
  Slot_fb3_R/1(data_h) -> data_fb3_R/1  "data_fb3_R"
  Slot_fb3_R/2(len_h) -> len_fb3_R/1  "len_fb3_R"
  Slot_fb3_R/3(cnt) -> cnt_fb3_R/1  "cnt_fb3_R"
  Slot_fb2_L/1(data_h) -> data_fb2_L/1  "data_fb2_L"
  Slot_fb2_L/2(len_h) -> len_fb2_L/1  "len_fb2_L"
  Slot_fb2_L/3(cnt) -> cnt_fb2_L/1  "cnt_fb2_L"
  Slot_fb2_R/1(data_h) -> data_fb2_R/1  "data_fb2_R"
  Slot_fb2_R/2(len_h) -> len_fb2_R/1  "len_fb2_R"
  Slot_fb2_R/3(cnt) -> cnt_fb2_R/1  "cnt_fb2_R"
  Slot_impl_fb/1(data_h) -> data_impl_fb/1  "data_impl_fb"
  Slot_impl_fb/2(len_h) -> len_impl_fb/1  "len_impl_fb"
  Slot_impl_fb/3(cnt) -> cnt_impl_fb/1  "cnt_impl_fb"
  Slot_limits/1(data_h) -> data_limits/1  "data_limits"
  Slot_limits/2(len_h) -> len_limits/1  "len_limits"
  Slot_limits/3(cnt) -> cnt_limits/1  "cnt_limits"
  Slot_soc/1(data_h) -> data_soc/1  "data_soc"
  Slot_soc/2(len_h) -> len_soc/1  "len_soc"
  Slot_soc/3(cnt) -> cnt_soc/1  "cnt_soc"
  Slot_vit/1(data_h) -> data_vit/1  "data_vit"
  Slot_vit/2(len_h) -> len_vit/1  "len_vit"
  Slot_vit/3(cnt) -> cnt_vit/1  "cnt_vit"
  Slot_alarm/1(data_h) -> data_alarm/1  "data_alarm"
  Slot_alarm/2(len_h) -> len_alarm/1  "len_alarm"
  Slot_alarm/3(cnt) -> cnt_alarm/1  "cnt_alarm"
  Slot_cells/1(data_h) -> data_cells/1  "data_cells"
  Slot_cells/2(len_h) -> len_cells/1  "len_cells"
  Slot_cells/3(cnt) -> cnt_cells/1  "cnt_cells"
  Slot_state/1(data_h) -> data_state/1  "data_state"
  Slot_state/2(len_h) -> len_state/1  "len_state"
  Slot_state/3(cnt) -> cnt_state/1  "cnt_state"
  Slot_power/1(data_h) -> data_power/1  "data_power"
  Slot_power/2(len_h) -> len_power/1  "len_power"
  Slot_power/3(cnt) -> cnt_power/1  "cnt_power"

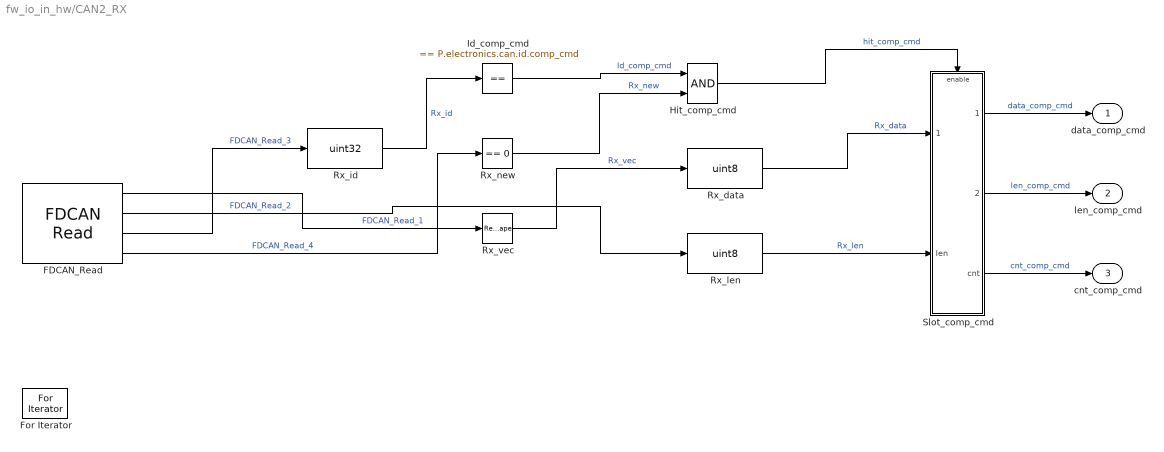
== system fw_io_in_hw/CAN2_RX ==
  FDCAN_Read : stm32blockslib/FDCAN Read  FDCANModule=FDCAN2  BlockMode=Receive  OperationReadMode=Data  OperationWriteMode=Data  ReadSource=FIFO 0  BufferNumber=0  OutputTypeReadMode=Unpacked  DataFormatWriteMode=Raw data  CANFrameType=CAN-FD  IdentifierTypeVia=Dialog  IdentifierType=Standard (11-bit identifier)  IdentifierVia=Inport  Identifier=100  DataLengthVia=Inport  DataLength=64  OutputIdType=off  IsBitRateSwitchingEnabled=off  TransmitRemoteFrame=off  OutputFrameType=off  OutputBRS=off  OutputRemoteFrame=off  OutputTxFifoLevel=off  OutputRxFifoLevel=off  OutputStatus=on  Timeout=0.001  SampleTime=-1
      settings: LibrarySourceBlock=stm32h7xxblockslib/FDCAN Read
  For Iterator : ForIterator  IterationLimit=P.electronics.hw.can2_rx_iter  ShowIterationPort=off
  Hit_comp_cmd : Logic  AllPortsSameDT=off  OutDataTypeStr=boolean
  Id_comp_cmd : simulink/Logic and Bit Operations/Compare To Constant  relop===  const=P.electronics.can.id.comp_cmd  OutDataTypeStr=boolean
  Rx_data : DataTypeConversion  OutDataTypeStr=uint8  RndMeth=Round
  Rx_id : DataTypeConversion  OutDataTypeStr=uint32  RndMeth=Round
  Rx_len : DataTypeConversion  OutDataTypeStr=uint8  RndMeth=Round
  Rx_new : simulink/Logic and Bit Operations/Compare To Zero  relop===  OutDataTypeStr=boolean
  Rx_vec : Reshape
  Slot_comp_cmd : Subsystem
  data_comp_cmd : Outport
  len_comp_cmd : Outport  Port=2
  cnt_comp_cmd : Outport  Port=3
  wires:
  FDCAN_Read/1 -> Rx_vec/1  "FDCAN_Read_1"
  FDCAN_Read/2 -> Rx_len/1  "FDCAN_Read_2"
  FDCAN_Read/3 -> Rx_id/1  "FDCAN_Read_3"
  FDCAN_Read/4 -> Rx_new/1  "FDCAN_Read_4"
  Rx_id/1 -> Id_comp_cmd/1  "Rx_id"
  Id_comp_cmd/1 -> Hit_comp_cmd/1  "Id_comp_cmd"
  Rx_new/1 -> Hit_comp_cmd/2  "Rx_new"
  Rx_vec/1 -> Rx_data/1  "Rx_vec"
  Hit_comp_cmd/1 -> Slot_comp_cmd/Enable  "hit_comp_cmd"
  Rx_data/1 -> Slot_comp_cmd/1(data)  "Rx_data"
  Rx_len/1 -> Slot_comp_cmd/2(len)  "Rx_len"
  Slot_comp_cmd/1(data_h) -> data_comp_cmd/1  "data_comp_cmd"
  Slot_comp_cmd/2(len_h) -> len_comp_cmd/1  "len_comp_cmd"
  Slot_comp_cmd/3(cnt) -> cnt_comp_cmd/1  "cnt_comp_cmd"

== system fw_io_in_hw/RMVF_write ==
  Enable : EnablePort
  RCC_RSR_RMVF : stmutilitieslib/Register Read//Write  Description=INTENDED (set in the T17 board setup): tgtHW 'STM32H7xx Based', devID 'STM32H743', regGrpName 'RCC', regName 'RSR', opCode 'Write'.  tgtHW=STM32F4xx Based  devID=STM32F401  regGrpName=ADC_Common  regName=CSR  accessMode=Specified bits  opCode=Read  bitsToBeProcessed={ [ 15, 0 ] }  bitFields={'on','All';'off','OVR3';'off','STRT3';'off','JSTRT3';'off','JEOC3';'off','EOC3';'off','AWD3';'off','OVR2';'off','STRT2';'off','JSTRT2';'off','JEOC2';'off','EOC2';'off','AWD2';'off','OVR1';'off','STRT1';'off','JSTRT1';'off','JEOC1';'off','EOC1';'off','AWD1'}  SampleTime=1
  RCC_RSR_RMVF_rd : Terminator
  RCC_RSR_RMVF_value : Terminator
  RMVF : Constant  Value=2^P.electronics.hw.rcc_rsr_rmvf_bit  OutDataTypeStr=uint32  SampleTime=-1
  wires:
  RMVF/1 -> RCC_RSR_RMVF_value/1  "RMVF"
  RCC_RSR_RMVF/1 -> RCC_RSR_RMVF_rd/1  "RCC_RSR_RMVF"

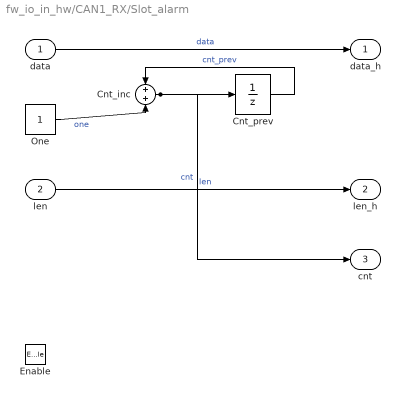
== system fw_io_in_hw/CAN1_RX/Slot_alarm ==
  data : Inport
  len : Inport  Port=2
  Enable : EnablePort
  Cnt_inc : Sum  OutDataTypeStr=uint8
  Cnt_prev : UnitDelay  SampleTime=-1
  One : Constant  OutDataTypeStr=uint8  SampleTime=-1
  data_h : Outport  InitialOutput=zeros(1,8)
  len_h : Outport  Port=2  InitialOutput=0
  cnt : Outport  Port=3  InitialOutput=0
  wires:
  data/1 -> data_h/1  "data"
  One/1 -> Cnt_inc/2  "one"
  len/1 -> len_h/1  "len"
  Cnt_inc/1 -> cnt/1, Cnt_prev/1  "cnt"
  Cnt_prev/1 -> Cnt_inc/1  "cnt_prev"

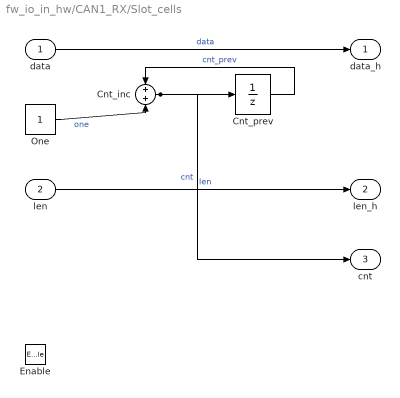
== system fw_io_in_hw/CAN1_RX/Slot_cells ==
  data : Inport
  len : Inport  Port=2
  Enable : EnablePort
  Cnt_inc : Sum  OutDataTypeStr=uint8
  Cnt_prev : UnitDelay  SampleTime=-1
  One : Constant  OutDataTypeStr=uint8  SampleTime=-1
  data_h : Outport  InitialOutput=zeros(1,8)
  len_h : Outport  Port=2  InitialOutput=0
  cnt : Outport  Port=3  InitialOutput=0
  wires:
  data/1 -> data_h/1  "data"
  One/1 -> Cnt_inc/2  "one"
  len/1 -> len_h/1  "len"
  Cnt_inc/1 -> cnt/1, Cnt_prev/1  "cnt"
  Cnt_prev/1 -> Cnt_inc/1  "cnt_prev"

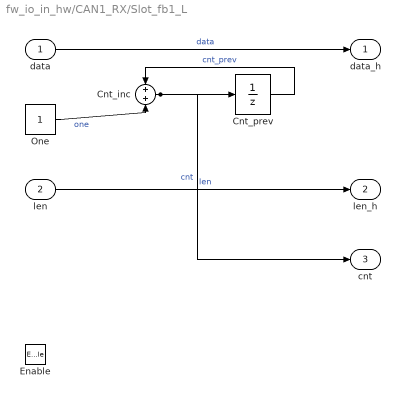
== system fw_io_in_hw/CAN1_RX/Slot_fb1_L ==
  data : Inport
  len : Inport  Port=2
  Enable : EnablePort
  Cnt_inc : Sum  OutDataTypeStr=uint8
  Cnt_prev : UnitDelay  SampleTime=-1
  One : Constant  OutDataTypeStr=uint8  SampleTime=-1
  data_h : Outport  InitialOutput=zeros(1,8)
  len_h : Outport  Port=2  InitialOutput=0
  cnt : Outport  Port=3  InitialOutput=0
  wires:
  data/1 -> data_h/1  "data"
  One/1 -> Cnt_inc/2  "one"
  len/1 -> len_h/1  "len"
  Cnt_inc/1 -> cnt/1, Cnt_prev/1  "cnt"
  Cnt_prev/1 -> Cnt_inc/1  "cnt_prev"

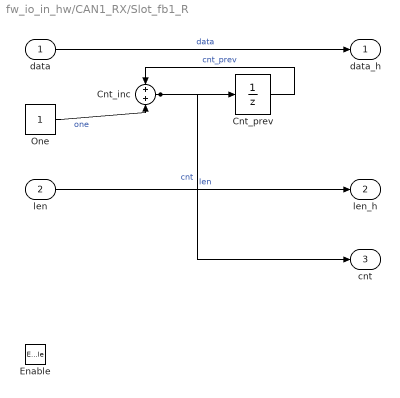
== system fw_io_in_hw/CAN1_RX/Slot_fb1_R ==
  data : Inport
  len : Inport  Port=2
  Enable : EnablePort
  Cnt_inc : Sum  OutDataTypeStr=uint8
  Cnt_prev : UnitDelay  SampleTime=-1
  One : Constant  OutDataTypeStr=uint8  SampleTime=-1
  data_h : Outport  InitialOutput=zeros(1,8)
  len_h : Outport  Port=2  InitialOutput=0
  cnt : Outport  Port=3  InitialOutput=0
  wires:
  data/1 -> data_h/1  "data"
  One/1 -> Cnt_inc/2  "one"
  len/1 -> len_h/1  "len"
  Cnt_inc/1 -> cnt/1, Cnt_prev/1  "cnt"
  Cnt_prev/1 -> Cnt_inc/1  "cnt_prev"

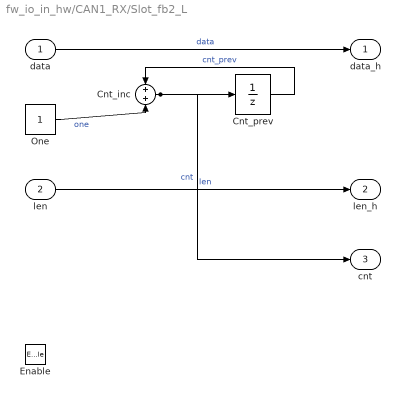
== system fw_io_in_hw/CAN1_RX/Slot_fb2_L ==
  data : Inport
  len : Inport  Port=2
  Enable : EnablePort
  Cnt_inc : Sum  OutDataTypeStr=uint8
  Cnt_prev : UnitDelay  SampleTime=-1
  One : Constant  OutDataTypeStr=uint8  SampleTime=-1
  data_h : Outport  InitialOutput=zeros(1,8)
  len_h : Outport  Port=2  InitialOutput=0
  cnt : Outport  Port=3  InitialOutput=0
  wires:
  data/1 -> data_h/1  "data"
  One/1 -> Cnt_inc/2  "one"
  len/1 -> len_h/1  "len"
  Cnt_inc/1 -> cnt/1, Cnt_prev/1  "cnt"
  Cnt_prev/1 -> Cnt_inc/1  "cnt_prev"

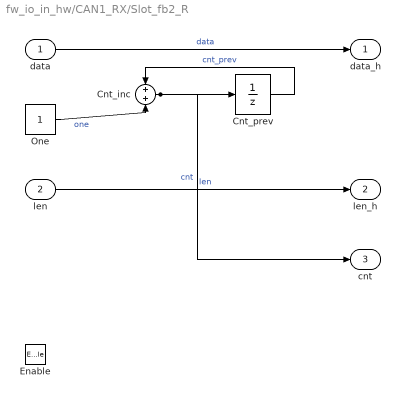
== system fw_io_in_hw/CAN1_RX/Slot_fb2_R ==
  data : Inport
  len : Inport  Port=2
  Enable : EnablePort
  Cnt_inc : Sum  OutDataTypeStr=uint8
  Cnt_prev : UnitDelay  SampleTime=-1
  One : Constant  OutDataTypeStr=uint8  SampleTime=-1
  data_h : Outport  InitialOutput=zeros(1,8)
  len_h : Outport  Port=2  InitialOutput=0
  cnt : Outport  Port=3  InitialOutput=0
  wires:
  data/1 -> data_h/1  "data"
  One/1 -> Cnt_inc/2  "one"
  len/1 -> len_h/1  "len"
  Cnt_inc/1 -> cnt/1, Cnt_prev/1  "cnt"
  Cnt_prev/1 -> Cnt_inc/1  "cnt_prev"

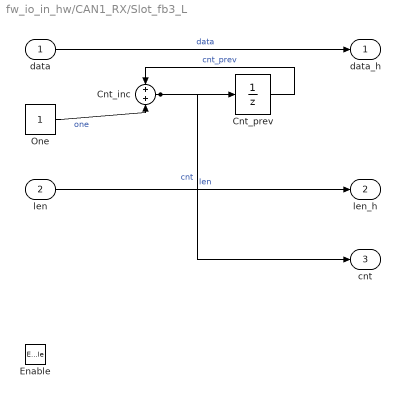
== system fw_io_in_hw/CAN1_RX/Slot_fb3_L ==
  data : Inport
  len : Inport  Port=2
  Enable : EnablePort
  Cnt_inc : Sum  OutDataTypeStr=uint8
  Cnt_prev : UnitDelay  SampleTime=-1
  One : Constant  OutDataTypeStr=uint8  SampleTime=-1
  data_h : Outport  InitialOutput=zeros(1,8)
  len_h : Outport  Port=2  InitialOutput=0
  cnt : Outport  Port=3  InitialOutput=0
  wires:
  data/1 -> data_h/1  "data"
  One/1 -> Cnt_inc/2  "one"
  len/1 -> len_h/1  "len"
  Cnt_inc/1 -> cnt/1, Cnt_prev/1  "cnt"
  Cnt_prev/1 -> Cnt_inc/1  "cnt_prev"

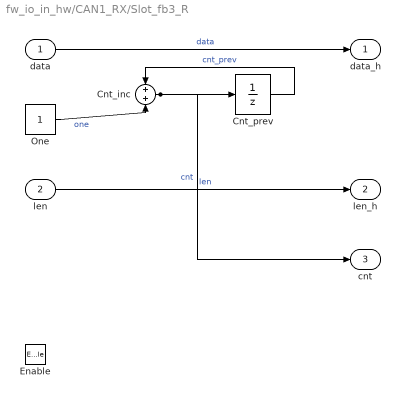
== system fw_io_in_hw/CAN1_RX/Slot_fb3_R ==
  data : Inport
  len : Inport  Port=2
  Enable : EnablePort
  Cnt_inc : Sum  OutDataTypeStr=uint8
  Cnt_prev : UnitDelay  SampleTime=-1
  One : Constant  OutDataTypeStr=uint8  SampleTime=-1
  data_h : Outport  InitialOutput=zeros(1,8)
  len_h : Outport  Port=2  InitialOutput=0
  cnt : Outport  Port=3  InitialOutput=0
  wires:
  data/1 -> data_h/1  "data"
  One/1 -> Cnt_inc/2  "one"
  len/1 -> len_h/1  "len"
  Cnt_inc/1 -> cnt/1, Cnt_prev/1  "cnt"
  Cnt_prev/1 -> Cnt_inc/1  "cnt_prev"

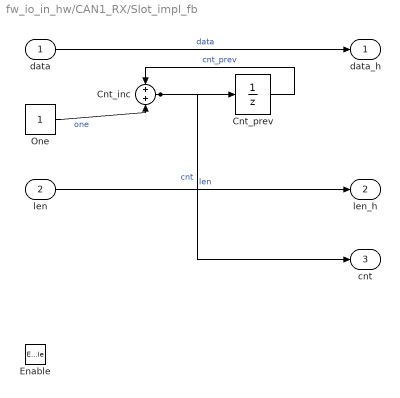
== system fw_io_in_hw/CAN1_RX/Slot_impl_fb ==
  data : Inport
  len : Inport  Port=2
  Enable : EnablePort
  Cnt_inc : Sum  OutDataTypeStr=uint8
  Cnt_prev : UnitDelay  SampleTime=-1
  One : Constant  OutDataTypeStr=uint8  SampleTime=-1
  data_h : Outport  InitialOutput=zeros(1,8)
  len_h : Outport  Port=2  InitialOutput=0
  cnt : Outport  Port=3  InitialOutput=0
  wires:
  data/1 -> data_h/1  "data"
  One/1 -> Cnt_inc/2  "one"
  len/1 -> len_h/1  "len"
  Cnt_inc/1 -> cnt/1, Cnt_prev/1  "cnt"
  Cnt_prev/1 -> Cnt_inc/1  "cnt_prev"

== system fw_io_in_hw/CAN1_RX/Slot_limits ==
  data : Inport
  len : Inport  Port=2
  Enable : EnablePort
  Cnt_inc : Sum  OutDataTypeStr=uint8
  Cnt_prev : UnitDelay  SampleTime=-1
  One : Constant  OutDataTypeStr=uint8  SampleTime=-1
  data_h : Outport  InitialOutput=zeros(1,8)
  len_h : Outport  Port=2  InitialOutput=0
  cnt : Outport  Port=3  InitialOutput=0
  wires:
  data/1 -> data_h/1  "data"
  One/1 -> Cnt_inc/2  "one"
  len/1 -> len_h/1  "len"
  Cnt_inc/1 -> cnt/1, Cnt_prev/1  "cnt"
  Cnt_prev/1 -> Cnt_inc/1  "cnt_prev"

== system fw_io_in_hw/CAN1_RX/Slot_power ==
  data : Inport
  len : Inport  Port=2
  Enable : EnablePort
  Cnt_inc : Sum  OutDataTypeStr=uint8
  Cnt_prev : UnitDelay  SampleTime=-1
  One : Constant  OutDataTypeStr=uint8  SampleTime=-1
  data_h : Outport  InitialOutput=zeros(1,8)
  len_h : Outport  Port=2  InitialOutput=0
  cnt : Outport  Port=3  InitialOutput=0
  wires:
  data/1 -> data_h/1  "data"
  One/1 -> Cnt_inc/2  "one"
  len/1 -> len_h/1  "len"
  Cnt_inc/1 -> cnt/1, Cnt_prev/1  "cnt"
  Cnt_prev/1 -> Cnt_inc/1  "cnt_prev"

== system fw_io_in_hw/CAN1_RX/Slot_soc ==
  data : Inport
  len : Inport  Port=2
  Enable : EnablePort
  Cnt_inc : Sum  OutDataTypeStr=uint8
  Cnt_prev : UnitDelay  SampleTime=-1
  One : Constant  OutDataTypeStr=uint8  SampleTime=-1
  data_h : Outport  InitialOutput=zeros(1,8)
  len_h : Outport  Port=2  InitialOutput=0
  cnt : Outport  Port=3  InitialOutput=0
  wires:
  data/1 -> data_h/1  "data"
  One/1 -> Cnt_inc/2  "one"
  len/1 -> len_h/1  "len"
  Cnt_inc/1 -> cnt/1, Cnt_prev/1  "cnt"
  Cnt_prev/1 -> Cnt_inc/1  "cnt_prev"

== system fw_io_in_hw/CAN1_RX/Slot_state ==
  data : Inport
  len : Inport  Port=2
  Enable : EnablePort
  Cnt_inc : Sum  OutDataTypeStr=uint8
  Cnt_prev : UnitDelay  SampleTime=-1
  One : Constant  OutDataTypeStr=uint8  SampleTime=-1
  data_h : Outport  InitialOutput=zeros(1,8)
  len_h : Outport  Port=2  InitialOutput=0
  cnt : Outport  Port=3  InitialOutput=0
  wires:
  data/1 -> data_h/1  "data"
  One/1 -> Cnt_inc/2  "one"
  len/1 -> len_h/1  "len"
  Cnt_inc/1 -> cnt/1, Cnt_prev/1  "cnt"
  Cnt_prev/1 -> Cnt_inc/1  "cnt_prev"

== system fw_io_in_hw/CAN1_RX/Slot_vit ==
  data : Inport
  len : Inport  Port=2
  Enable : EnablePort
  Cnt_inc : Sum  OutDataTypeStr=uint8
  Cnt_prev : UnitDelay  SampleTime=-1
  One : Constant  OutDataTypeStr=uint8  SampleTime=-1
  data_h : Outport  InitialOutput=zeros(1,8)
  len_h : Outport  Port=2  InitialOutput=0
  cnt : Outport  Port=3  InitialOutput=0
  wires:
  data/1 -> data_h/1  "data"
  One/1 -> Cnt_inc/2  "one"
  len/1 -> len_h/1  "len"
  Cnt_inc/1 -> cnt/1, Cnt_prev/1  "cnt"
  Cnt_prev/1 -> Cnt_inc/1  "cnt_prev"

== system fw_io_in_hw/CAN2_RX/Slot_comp_cmd ==
  data : Inport
  len : Inport  Port=2
  Enable : EnablePort
  Cnt_inc : Sum  OutDataTypeStr=uint8
  Cnt_prev : UnitDelay  SampleTime=-1
  One : Constant  OutDataTypeStr=uint8  SampleTime=-1
  data_h : Outport  InitialOutput=zeros(1,64)
  len_h : Outport  Port=2  InitialOutput=0
  cnt : Outport  Port=3  InitialOutput=0
  wires:
  data/1 -> data_h/1  "data"
  One/1 -> Cnt_inc/2  "one"
  len/1 -> len_h/1  "len"
  Cnt_inc/1 -> cnt/1, Cnt_prev/1  "cnt"
  Cnt_prev/1 -> Cnt_inc/1  "cnt_prev"
